simulink model "Sim_Electromecanico"  (R2026a)
settings: Solver=VariableStepAuto  StopTime=5
InitFcn:
  | Vin = 5;
  | Ra = 2;
  | La = 23e-3;
  | Ke = 10e-3;
  | Kt = 10e-3;
  | J = 1e-3;
  | b = 1.2e-3;
libraries: fl_lib x9, nesl_utility x2
settings Model: Creator=jair  LastModifiedBy=Jaras

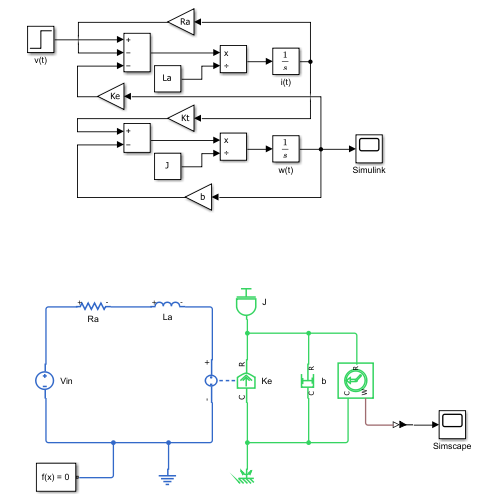
[thumbnail: Simulink's stored preview of the top-level diagram]
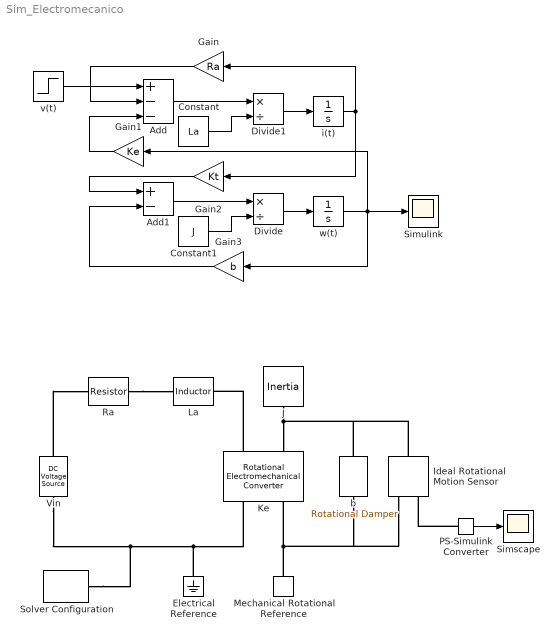
== system Sim_Electromecanico ==
  Add : Sum  Inputs=+--
  Add1 : Sum  Inputs=+-
  Constant : Constant  Value=La
  Constant1 : Constant  Value=J
  Divide : Product  Inputs=*/
  Divide1 : Product  Inputs=*/
  Electrical Reference : fl_lib/Electrical/Electrical Elements/Electrical Reference
  Gain : Gain  Gain=Ra
  Gain1 : Gain  Gain=Ke
  Gain2 : Gain  Gain=Kt
  Gain3 : Gain  Gain=b
  Ideal Rotational Motion Sensor : fl_lib/Mechanical/Mechanical Sensors/Ideal Rotational Motion Sensor  reference=foundation.enum.MeasurementReference.difference  acceleration_port=false  velocity_port=true  position_port=false  wrap_angle=false  offset=0 rad
  J : fl_lib/Mechanical/Rotational Elements/Inertia  inertia=J kg*m^2  num_ports=foundation.enum.numPorts2.one  w_specify=off  w_priority=High  w=0 rad/s  w_nominal_specify=off  w_nominal_value=1  w_nominal_unit=rad/s  t_specify=off  t_priority=None  t=0 N*m  t_nominal_specify=off  t_nominal_value=1  t_nominal_unit=N*m
  Ke : fl_lib/Electrical/Electrical Elements/Rotational Electromechanical Converter  K=Ke V*s/rad  i_specify=off  i_priority=None  i=0 A  i_nominal_specify=off  i_nominal_value=1  i_nominal_unit=A  v_specify=off  v_priority=None  v=0 V  v_nominal_specify=off  v_nominal_value=1  v_nominal_unit=V  t_specify=off  t_priority=None  t=0 N*m  t_nominal_specify=off  t_nominal_value=1  t_nominal_unit=N*m  w_specify=off  w_priority=None  w=0 rad/s  w_nominal_specify=off  w_nominal_value=1  w_nominal_unit=rad/s
  La : fl_lib/Electrical/Electrical Elements/Inductor  l=La H  r=0 Ohm  g=0 1/Ohm  i_specify=off  i_priority=None  i=0 A  i_nominal_specify=off  i_nominal_value=1  i_nominal_unit=A  v_specify=off  v_priority=None  v=0 V  v_nominal_specify=off  v_nominal_value=1  v_nominal_unit=V  i_L_specify=off  i_L_priority=High  i_L=0 A  i_L_nominal_specify=off  i_L_nominal_value=1  i_L_nominal_unit=A
  Mechanical Rotational Reference : fl_lib/Mechanical/Rotational Elements/Mechanical Rotational Reference
  PS-Simulink Converter : nesl_utility/PS-Simulink Converter  PhysicalDomain=network_engine_domain  SubClassName=ps_output  LeftPortType=input  RightPortType=output  PseudoPeriodic=off  Frequencies=[]  VectorFormat=inherit  Unit=inherit  AffineConversion=off
  Ra : fl_lib/Electrical/Electrical Elements/Resistor  R=Ra Ohm  i_specify=off  i_priority=None  i=0 A  i_nominal_specify=off  i_nominal_value=1  i_nominal_unit=A  v_specify=off  v_priority=None  v=0 V  v_nominal_specify=off  v_nominal_value=1  v_nominal_unit=V
  Simscape : Scope
      settings: ActiveDisplayYMinimum=-2.4951237985135211  ActiveDisplayYMaximum=22.456114186621694
  Simulink : Scope
      settings: ActiveDisplayYMinimum=-2.495123798513522  ActiveDisplayYMaximum=22.4561141866217
  Solver Configuration : nesl_utility/Solver Configuration  PhysicalDomain=network_engine_domain  SubClassName=solver  LeftPortType=input  RightPortType=generic  Tones=[]  Harmonics=[]  SimulateNoise=off  Profile=off  UseLocalSampling=off  EnableSwitchedLinearOptims=on  FrequencyDomain=off  UseCCode=off  RelTol=0.001  AbsTol=0.001  MinStep=1e-09  ToWorkspace=off  RevertToSquareIcSolve=off  NumHomotopyIterations=100  PhasorMode=off  PhasorModeNumHarmonics=1  ConsistencySolver=NEWTON_XTOL_AFTER_FTOL  CanonicalOrdering=CANONICAL  OptimizeIntermediates=OPTIMIZED  IndexReductionMethod=DerivativeReplacement  DoDC=off  ResidualTolerance=1e-09  ConsistencyTolSource=GLOBAL  ConsistencyAbsTol=0.001  ConsistencyRelTol=0.001  ConsistencyTolFactor=0.001  UseLocalSolver=off  LocalSolverChoice=NE_BACKWARD_EULER_ADVANCER  ResolveIndetEquations=on  FunctionEvalNumThread=1  LocalSolverSampleTime=0.001  DoFixedCost=off  MaxNonlinIter=3  MaxModeIter=2  ComputeImpulses=off  ImpulseIterations=2  LinearAlgebra=auto  LinearAlgebraNumThread=0  EquationFormulation=NE_TIME_EF  DelaysMemoryBudget=1024  AutomaticFiltering=on  FilteringTimeConstant=0.001  PartitionStorageMethod=AS_NEEDED  PartitionMemoryBudget=1024  PartitionMethod=ROBUST  MultibodyUseLocalSolver=off  MultibodyLocalSolverChoice=ODE1  MultibodyLocalSolverSampleTime=0.001
  Vin : fl_lib/Electrical/Electrical Sources/DC Voltage Source  v0=Vin V
  b : fl_lib/Mechanical/Rotational Elements/Rotational Damper  D=b N*m*s/rad  w_specify=off  w_priority=None  w=0 rad/s  w_nominal_specify=off  w_nominal_value=1  w_nominal_unit=rad/s  t_specify=off  t_priority=None  t=0 N*m  t_nominal_specify=off  t_nominal_value=1  t_nominal_unit=N*m
  i(t) : Integrator
  v(t) : Step  Time=0  FinalValue=Vin  SampleTime=0
  w(t) : Integrator
  wires:
  PS-Simulink Converter/1 -> Simscape/1
  Divide/1 -> w(t)/1
  Divide1/1 -> i(t)/1
  Constant/1 -> Divide1/2
  Constant1/1 -> Divide/2
  Add1/1 -> Divide/1
  Add/1 -> Divide1/1
  i(t)/1 -> Gain/1, Gain2/1
  Gain/1 -> Add/2
  w(t)/1 -> Simulink/1, Gain3/1, Gain1/1
  Gain1/1 -> Add/3
  Gain2/1 -> Add1/1
  Gain3/1 -> Add1/2
  v(t)/1 -> Add/1
  connections:
  Ke/LConn1 -- La/RConn1
  Ra/RConn1 -- La/LConn1
  Vin/LConn1 -- Ra/LConn1
  Vin/RConn1 -- Solver Configuration/RConn1 -- Electrical Reference/LConn1 -- Ke/RConn1
  J/LConn1 -- Ideal Rotational Motion Sensor/LConn1 -- b/LConn1 -- Ke/LConn2
  Mechanical Rotational Reference/LConn1 -- Ideal Rotational Motion Sensor/RConn1 -- b/RConn1 -- Ke/RConn2
  PS-Simulink Converter/LConn1 -- Ideal Rotational Motion Sensor/RConn2
